simulink model "demo_sti"  (R2026a)
settings: Solver=VariableStepAuto  StopTime=10
libraries: sharedtransform x1, mfeval_LIB x1
Description:
  | Copyright 2020-2024 The MathWorks, Inc.
settings Model: Creator=MFURLANT  LastModifiedBy=andrei

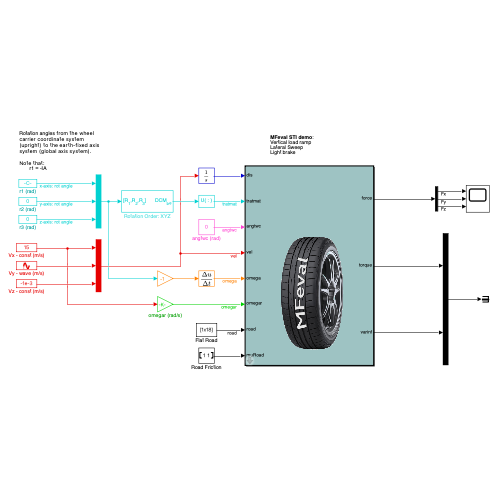
[thumbnail: Simulink's stored preview of the top-level diagram]
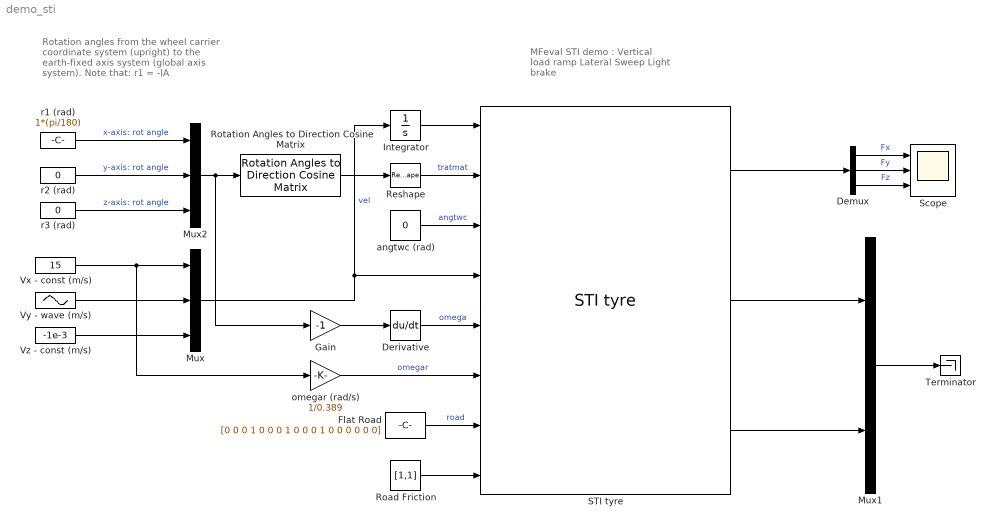
== system demo_sti ==
  note: MFeval STI demo :
      | Vertical load ramp
      | Lateral Sweep
      | Light brake
  note: Rotation angles from the wheel carrier coordinate system (upright) to the earth-fixed axis system (global axis system).
      |
      | Note that:
      | r1 = -IA
  Demux : Demux  Outputs=3
  Derivative : Derivative
  Flat Road : Constant  Value=[0 0 0 1 0 0 0 1 0 0 0 1 0 0 0 0 0 0]
  Gain : Gain  Gain=-1
  Integrator : Integrator  InitialCondition=0.38
  Mux : Mux  Inputs=3
  Mux1 : Mux  Inputs=2
  Mux2 : Mux  Inputs=3
  Reshape : Reshape
  Road Friction : Constant  Value=[1,1]
  Rotation Angles to Direction Cosine Matrix : sharedtransform/Rotation Angles to Direction Cosine Matrix  rotationOrder=XYZ  aMode=aMode
  STI tyre : mfeval_LIB/STI tyre  Description=Magic Formula 6.1.2 tyre model including relaxation length and transient calculations  userParameterSource='MagicFormula61_Paramerters.tir'  userSide=1 left  userDynamics=2 linear transients  userUseMode=1 combined  enablePressure=off  userPressure=2.3
      settings: SourceProductName=MFeval Library
  Scope : Scope  NumInputPorts=3
      settings: ActiveDisplayYMinimum=-4372.01549  ActiveDisplayYMaximum=385.11185
  Terminator : Terminator
  Vx - const (m/s) : Constant  Value=15
  Vy - wave (m/s) : Sin  Amplitude=0.1  SampleTime=0
  Vz - const (m/s) : Constant  Value=-1e-3
  angtwc (rad) : Constant  Value=0
  omegar (rad/s) : Gain  Gain=1/0.389
  r1 (rad) : Constant  Value=1*(pi/180)
  r2 (rad) : Constant  Value=0
  r3 (rad) : Constant  Value=0
  wires:
  Reshape/1 -> STI tyre/2  "tratmat"
  Derivative/1 -> STI tyre/5  "omega"
  Mux/1 -> Integrator/1, STI tyre/4  "vel"
  angtwc (rad)/1 -> STI tyre/3  "angtwc"
  Vz - const (m/s)/1 -> Mux/3
  omegar (rad/s)/1 -> STI tyre/6  "omegar"
  Vy - wave (m/s)/1 -> Mux/2
  Vx - const (m/s)/1 -> Mux/1, omegar (rad/s)/1
  Flat Road/1 -> STI tyre/7  "road"
  Mux1/1 -> Terminator/1
  STI tyre/3 -> Mux1/2
  STI tyre/2 -> Mux1/1
  STI tyre/1 -> Demux/1
  Road Friction/1 -> STI tyre/8
  Integrator/1 -> STI tyre/1
  Rotation Angles to Direction Cosine Matrix/1 -> Reshape/1
  r2 (rad)/1 -> Mux2/2  "y-axis: rot angle"
  r3 (rad)/1 -> Mux2/3  "z-axis: rot angle"
  r1 (rad)/1 -> Mux2/1  "x-axis: rot angle"
  Demux/1 -> Scope/1  "Fx"
  Demux/2 -> Scope/2  "Fy"
  Demux/3 -> Scope/3  "Fz"
  Mux2/1 -> Gain/1, Rotation Angles to Direction Cosine Matrix/1
  Gain/1 -> Derivative/1
